simulink model "XFLUID04_reference"  (R2025a)
settings: Solver=ode23t  StartTime=0  StopTime=20  MaxStep=0.02  RelTol=1e-3  AbsTol=1e-4  EnableMultiTasking=on
PreLoadFcn:
  | warning('off','Simulink:Commands:LoadMdlParameterizedLink');
PostLoadFcn:
  | warning off sm:compiler:topologyAnalysis:DanglingBlock
  | warning off Simulink:SL_SolverMaskedZC;
  | warning off Simulink:SL_SolverIgnoredZCBracketing;
  | warning off Simulink:Engine:SolverMinStepNonlinearIterWarnForDAE;
  | warning off simscape:compiler:sli:init:SolverNotRecommended
  | warning off Simulink:Engine:UsingDiscreteSolver
  | warning('off','sm:sli:setup:compile:LocalSolverNotSupported')
  | warning off physmod:simscape:compiler:sli:init:SolverNotRecommended
  | warning off sm:sli:visualization:ModelRefNotSupported
  | warning off Simulink:modelReference:ProtectedModelCallbackLostWarning
StartFcn:
  | tic;
StopFcn:
  | Elapsed_Sim_Time = toc;
  | disp(['Elapsed Sim Time = ' num2str(Elapsed_Sim_Time)]);
undefined symbols (not defined in the file): actuator_hs_b, actuator_hs_k, lift_target_mm, Local, motion_start_s, motor_damping, pressure_step_offset_s, ramp_duration_s, Scissor_Lift_Param, supply_pressure_bar, supply_pressure_step_fraction, target_hold_s, X, Y, Z
libraries: fl_lib x108, sm_lib x41, Scissor_Parts_Lib x24, nesl_utility x9, SimscapeFluids_lib x2, Custom_lib x2, slpidlib x1, fl_ps_legacy_lib x1, simulink x1, ee_lib x1, Motor_Lib x1, sdl_lib x1
(part 1 of 3)
Description:
  | Copyright 2015-2025 The MathWorks, Inc.
settings Model: ExtModeTrigDuration=500  Creator=smiller  LastModifiedBy=SimuVerity Contributors
settings SolverCC: AutoScaleAbsTol=off  AlgebraicLoopSolver=TrustRegion  PositivePriorityOrder=on
settings DataIOCC: SaveFormat=Array
settings OptimizationCC: BlockReduction=off  OptimizeBlockIOStorage=off  BufferReuse=off  ReuseModelBlockBuffer=off  GlobalBufferReuse=off  ExpressionFolding=off  ExpressionDepthLimit=2147483647.0  LocalBlockOutputs=off  ZeroExternalMemoryAtStartup=off  ZeroInternalMemoryAtStartup=off  OptimizeDataStoreBuffers=off  BusAssignmentInplaceUpdate=off
settings DebuggingCC: UnderspecifiedInitializationDetection=Classic  MergeDetectMultiDrivingBlocksExec=none  UnconnectedInputMsg=warning  UnconnectedOutputMsg=warning  UnconnectedLineMsg=warning  AllowSymbolicDim=off  StateNameClashWarn=warning  PregeneratedLibrarySubsystemCodeDiagnostic=none  SFUnexpectedBacktrackingDiag=warning  SFNoUnconditionalDefaultTransitionDiag=warning  SFExecutionAtInitializationDiag=none  ArithmeticOperatorsInVariantConditions=warning
settings ModelReferenceCC: EnableRefExpFcnMdlSchedulingChecks=on  PropagateSignalLabelsOutOfModel=off
settings SFSimCC: SimUseLocalCustomCode=off  CustomCodeUndefinedFunction=UseInterfaceOnly
settings RTWCC: RTWUseLocalCustomCode=off  Toolchain=Simulink Real-Time Toolchain  BuildConfiguration=Faster Runs  TargetLang=C++  GPUComputeCapability=3.5  DLArmComputeVersion=19.05
settings CodeAppCC: StateflowObjectComments=on
settings GRTTargetCC: TargetLangStandard=C++03 (ISO)  CodeInterfacePackaging=C++ class
settings ConfigComp: CovMetricSettings=dw  CovSaveCumulativeToWorkspaceVar=on  CovSaveSingleToWorkspaceVar=on  CovExternalEMLEnable=off  CovSFcnEnable=off
settings SimscapeCC: ExplicitSolverDiagnosticOptions=none  SimscapeNormalizeSystem=off  SimscapeLogType=all  SimscapeLogSimulationStatistics=on  SimscapeLogName=simlog_ssc_hydraulic_lift  SimscapeLogLimitData=off
settings ConfigurationSet: Description=SimMechanics 2G
settings DiagnosticsConfigSet: SimMechanicsUnconnectedFramePorts=none
settings ExplorerConfigSet: SimMechanicsOpenEditorOnUpdate=off  InternalSimMechanicsExplorerSettings="<ExplorerConfiguration><canonicalview>default</canonicalview><AnimationSetting><BasePlaybackSpeed>1.0</BasePlaybackSpeed><PlaybackSpeedFactor>1.0</PlaybackSpeedFactor></AnimationSetting><TilePanel><TileInfo><Tiles Columns=\"1\" Count=\"1\" Rows=\"1\"><Column Left=\"2\" Weight=\"1\"/><Column Left=\"550\"/><Row Top=\"2\" Weight=\"1\"/><Row Top=\"610\"/><Tile Height=\"1\" Width=\"1\" X=\"0\" Y=\"0\"/></Tiles></TileInfo><SceneInfo><SceneViewer><BGColor><R>0.90980392694473267</R><G>1</G><B>1</B></BGColor><Camera><Position><X>-3.0625353892662139</X><Y>-4.5689256897751696</Y><Z>1.9819473078285381</Z></Position><Center><X>-0.9000098372499532</X><Y>-2.432211148661878e-05</Y><Z>1.1621088702953468</Z></Center><Up><X>0.060248240113841743</X><Y>0.14860062570234261</Y><Z>0.98706028367271337</Z></Up><Left>-1.3650000751018525</Left><Right>1.3650000751018525</Right><Bottom>-1.2464621901512147</Bottom><Top>1.2464621901512147</Top></Camera></SceneViewer></SceneInfo></TilePanel></ExplorerConfiguration>"

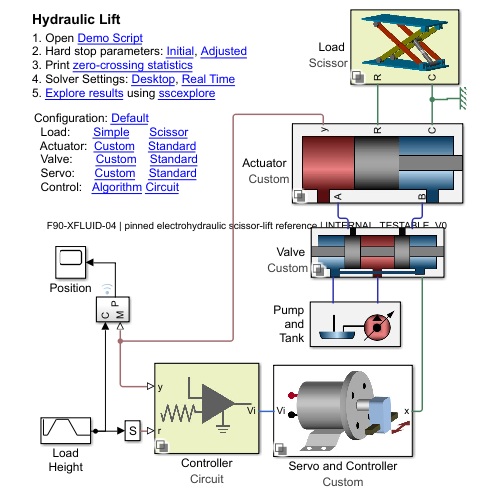
[thumbnail: Simulink's stored preview of the top-level diagram]
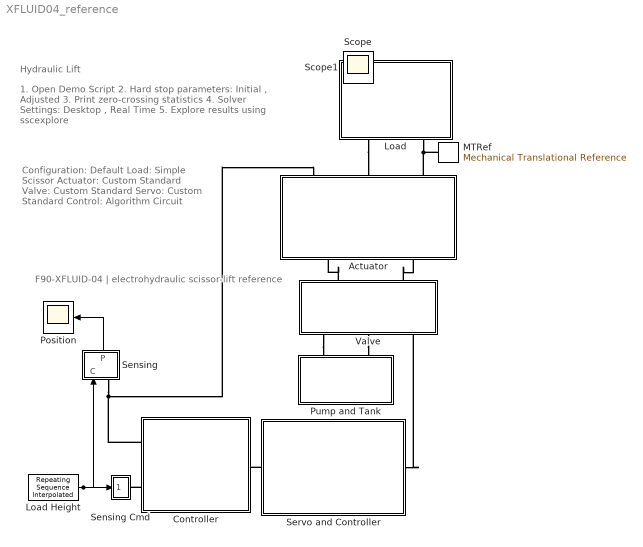
== system XFLUID04_reference ==
  note: Hydraulic Lift
  note: 1. Open Demo Script
      | 2. Hard stop parameters: Initial , Adjusted
      | 3. Print zero-crossing statistics
      | 4. Solver Settings: Desktop , Real Time
      | 5. Explore results using sscexplore
  note: Configuration: Default
      | Load: Simple Scissor
      | Actuator: Custom Standard
      | Valve: Custom Standard
      | Servo: Custom Standard
      | Control: Algorithm Circuit
  note: F90-XFLUID-04 | electrohydraulic scissor-lift reference
  Actuator : Subsystem  Variant=on  VariantControlMode=label  LabelModeActiveChoice=Custom
      settings: AttributesFormatString=%<ActiveVariant>
      mask Display:
      | blk = ssc_hydraulic_lift_activeVariantBlock(gcb);
      | eval(get_param(blk, 'MaskDisplay'));
  Controller : Subsystem  Variant=on  VariantControlMode=label  LabelModeActiveChoice=Circuit
      settings: AttributesFormatString=%<ActiveVariant>
      mask Display:
      | blk = ssc_hydraulic_lift_activeVariantBlock(gcb);
      | eval(get_param(blk, 'MaskDisplay'));
  Load : Subsystem  Variant=on  VariantControlMode=label  LabelModeActiveChoice=Scissor
      settings: AttributesFormatString=%<ActiveVariant>
      mask Display:
      | blk = ssc_hydraulic_lift_activeVariantBlock(gcb);
      | eval(get_param(blk, 'MaskDisplay'));
  Load Height : simulink/Sources/Repeating Sequence Interpolated  OutValues=[2.5 2.5 2.5+(lift_target_mm-50)*Scissor_Lift_Param.Sensor_Gain/1000 2.5+(lift_target_mm-50)*Scissor_Lift_Param.Sensor_Gain/1000 2.5 2.5]  TimeValues=[0 motion_start_s motion_start_s+ramp_duration_s motion_start_s+ramp_duration_s+target_hold_s motion_start_s+2*ramp_duration_s+target_hold_s 20]  LookUpMeth=Interpolation-Use End Values  tsamp=0.01  OutMin=[]  OutMax=[]  OutDataTypeStr=double  OutputDataTypeScalingMode=double  OutDataType=fixdt(0,8)  OutScaling=2^-10
  MTRef : fl_lib/Mechanical/Translational Elements/Mechanical Translational Reference
  Position : Scope
      settings: ActiveDisplayYMinimum=-77.71015  ActiveDisplayYMaximum=177.54113  DataLoggingVariableName=LoadPosition_DATA
  Pump and Tank : Subsystem
      mask Display: image('Pump_IMAGE.jpg');
  Sensing : Subsystem
  Sensing Cmd : Subsystem
      mask Display: disp('S')
  Servo and Controller : Subsystem  Variant=on  VariantControlMode=label  LabelModeActiveChoice=Custom
      settings: AttributesFormatString=%<ActiveVariant>
      mask Display:
      | blk = ssc_hydraulic_lift_activeVariantBlock(gcb);
      | eval(get_param(blk, 'MaskDisplay'));
  Valve : Subsystem  Variant=on  VariantControlMode=label  LabelModeActiveChoice=Custom
      settings: AttributesFormatString=%<ActiveVariant>
      mask Display:
      | blk = ssc_hydraulic_lift_activeVariantBlock(gcb);
      | eval(get_param(blk, 'MaskDisplay'));
  Scope : Scope
      settings: ActiveDisplayYMinimum=-0.84217  ActiveDisplayYMaximum=5.75412
  Scope1 : Scope
      settings: ActiveDisplayYMinimum=-0.31315  ActiveDisplayYMaximum=0.39292  DataLoggingVariableName=ScopeData2
  wires:
  Sensing/1(P) -> Position/1
  Load Height/1 -> Sensing/1(C), Sensing Cmd/1(In1)
  connections:
  MTRef/LConn1 -- Load/LConn2 -- Actuator/RConn3
  Valve/RConn1 -- Actuator/LConn1
  Valve/RConn2 -- Actuator/LConn2
  Controller/LConn1 -- Sensing/LConn1 -- Actuator/RConn1
  Load/LConn1 -- Actuator/RConn2
  Valve/LConn1 -- Pump and Tank/RConn1
  Valve/LConn2 -- Pump and Tank/RConn2
  Servo and Controller/RConn1 -- Valve/LConn3
  Servo and Controller/LConn1 -- Controller/RConn1
  Controller/LConn2 -- Sensing Cmd/RConn1

== system XFLUID04_reference/Actuator ==
  note: Variant Subsystem
  Custom : Subsystem  VariantControl=Custom  mask(Double-Acting Hydraulic Actuator){A=5e-4, V=10e-5, PA=200, PB=0, T=200, hs_k=actuator_hs_k, hs_b=actuator_hs_b}
      mask prompts: A "Piston area (m^2)"; V "Chamber dead volume (m^3)"; PA "Chamber A initial pressure (bar)"; PB "Chamber B initial pressure (bar)"; T "Piston travel (mm)"; hs_k "Hardstop stiffness (N/m)"; hs_b "Hardstop damping (N/(m/s))"
      mask help: Models a double-acting hydraulic actuator using Simscape Foundation library components.
      mask Display: image('Double_Acting_Cylinder_Custom_IMAGE.jpg');
  Standard : Subsystem  VariantControl=Standard  mask(Double-Acting Hydraulic Actuator){A=5e-4, V=10e-5, PA=200, PB=0, T=200, hs_k=actuator_hs_k, hs_b=actuator_hs_b}
      mask prompts: A "Piston area (m^2)"; V "Chamber dead volume (m^3)"; PA "Chamber A initial pressure (bar)"; PB "Chamber B initial pressure (bar)"; T "Piston travel (mm)"; hs_k "Hardstop stiffness (N/m)"; hs_b "Hardstop damping (N/(m/s))"
      mask help: Models a double-acting hydraulic actuator using Simscape add-on library components.
      mask Display: image('Double_Acting_Cylinder_Standard_IMAGE.jpg');
  A : PMIOPort  Side=Left
  B : PMIOPort  Port=2  Side=Left
  y : PMIOPort  Port=3  Side=Right
  R : PMIOPort  Port=4  Side=Right
  C : PMIOPort  Port=5  Side=Right

== system XFLUID04_reference/Controller ==
  Algorithm : Subsystem  VariantControl=Algorithm
      mask Display: image('Algorithm_Controller_IMAGE.jpg')
  Circuit : Subsystem  VariantControl=Circuit
      mask Display: image('Analog_PI_Controller_IMAGE.jpg')
  y : PMIOPort  Tag=PMCPort  Side=Left
  r : PMIOPort  Tag=PMCPort  Port=2  Side=Left
  Vi : PMIOPort  Port=3  Side=Right

== system XFLUID04_reference/Load ==
  Scissor : Subsystem  VariantControl=Scissor
      mask Display: image('Load_Scissor_IMAGE.jpg');
  Simple : Subsystem  VariantControl=Simple
      mask Display: image('Load_Simple_IMAGE.jpg');
  R : PMIOPort  Side=Left
  C : PMIOPort  Port=2  Side=Left

== system XFLUID04_reference/Pump and Tank ==
  Custom Hydraulic Fluid : fl_lib/Isothermal Liquid/Utilities/Isothermal Liquid Properties (IL)  rho_L_atm=850 kg/m^3  bulk_modulus_model=foundation.enum.bulk_modulus_model.const  beta_gain=6  beta_L_atm=8e+08 Pa  nu_atm=1.8e-05 m^2/s  p_atm=0.101325 MPa  p_min=1 Pa  properties_range_check=simscape.enum.assert.action.error  air_fraction=0.005  polytropic_index=1.0  rho_g_atm=1.225 kg/m^3  air_dissolution_model=false  p_crit=3 MPa
      settings: LibrarySourceBlock=fl_lib/Isothermal Liquid/Utilities/Isothermal Liquid Properties (IL)
  Hydraulic Reference : fl_lib/Isothermal Liquid/Elements/Reservoir (IL)  reservoir_type=foundation.enum.constant_controlled.constant  pressure_spec=foundation.enum.pressure_spec.atmospheric  reservoir_pressure=0.101325 MPa
  Pump : fl_lib/Isothermal Liquid/Sources/Pressure Source (IL)  source_type=foundation.enum.constant_controlled.controlled  pressure_differential=0 MPa
      settings: InternalSimscapePortConfiguration="{\"Bottom\":[],\"Left\":[{\"id\":\"A\",\"label\":\"A\",\"type\":\"foundation.isothermal_liquid.isothermal_liquid\"},{\"id\":\"P\",\"label\":\"P\",\"type\":\"input\"}],\"Right\":[{\"id\":\"B\",\"label\":\"B\",\"type\":\"foundation.isothermal_liquid.isothermal_liquid\"}],\"Top\":[]}"
  Solver Configuration : nesl_utility/Solver Configuration  PhysicalDomain=network_engine_domain  SubClassName=solver  LeftPortType=input  RightPortType=generic  Tones=[]  Harmonics=[]  SimulateNoise=off  Profile=off  UseLocalSampling=off  EnableSwitchedLinearOptims=on  FrequencyDomain=off  UseCCode=off  RelTol=0.001  AbsTol=1e-06  MinStep=1e-09  ToWorkspace=off  RevertToSquareIcSolve=off  NumHomotopyIterations=100  PhasorMode=off  PhasorModeNumHarmonics=1  ConsistencySolver=NEWTON_FTOL  IndexReductionMethod=DerivativeReplacement  DoDC=off  ResidualTolerance=1e-9  ConsistencyTolSource=GLOBAL  ConsistencyAbsTol=0.001  ConsistencyRelTol=0.001  ConsistencyTolFactor=0.001  UseLocalSolver=off  LocalSolverChoice=NE_BACKWARD_EULER_ADVANCER  ResolveIndetEquations=on  FunctionEvalNumThread=1  LocalSolverSampleTime=0.002  DoFixedCost=off  MaxNonlinIter=4  MaxModeIter=2  ComputeImpulses=off  ImpulseIterations=2  LinearAlgebra=Sparse  LinearAlgebraNumThread=0  EquationFormulation=NE_TIME_EF  DelaysMemoryBudget=1024  AutomaticFiltering=on  FilteringTimeConstant=0.001  PartitionStorageMethod=AS_NEEDED  PartitionMemoryBudget=1024  PartitionMethod=FAST  MultibodyUseLocalSolver=off  MultibodyLocalSolverChoice=ODE1  MultibodyLocalSolverSampleTime=0.001
  Supply Pressure : Step  Time=motion_start_s+ramp_duration_s+pressure_step_offset_s  Before=supply_pressure_bar  After=supply_pressure_bar*(1+supply_pressure_step_fraction)  SampleTime=0
  bar : nesl_utility/Simulink-PS Converter  PhysicalDomain=network_engine_domain  SubClassName=ps_input  LeftPortType=input  RightPortType=output  PseudoPeriodic=off  Frequencies=[]  NoiseDistribution=none  NoiseParameters=[]  Unit=bar  AffineConversion=off  FilteringAndDerivatives=zero  SimscapeFilterOrder=1  InputFilterTimeConstant=0.005  UdotUserProvided=0
  T : PMIOPort  Side=Right
  P : PMIOPort  Port=2  Side=Right
  wires:
  Supply Pressure/1 -> bar/1
  connections:
  Custom Hydraulic Fluid/RConn1 -- Solver Configuration/RConn1 -- T/RConn1 -- Pump/LConn1 -- Hydraulic Reference/LConn1
  P/RConn1 -- Pump/RConn1
  bar/RConn1 -- Pump/LConn2

== system XFLUID04_reference/Sensing ==
  C : Inport
  Fcn : Fcn  Expr=(u(1)-2.5)*1000/Scissor_Lift_Param.Sensor_Gain+50
  Mux : Mux  Inputs=2
  PS-Simulink Converter : nesl_utility/PS-Simulink Converter  PhysicalDomain=network_engine_domain  SubClassName=ps_output  LeftPortType=input  RightPortType=output  PseudoPeriodic=off  Frequencies=[]  VectorFormat=1-D array  Unit=mm  AffineConversion=off
  M : PMIOPort  Side=Left
  P : Outport  VectorParamsAs1DForOutWhenUnconnected=off
  wires:
  PS-Simulink Converter/1 -> Mux/2
  Mux/1 -> P/1
  Fcn/1 -> Mux/1
  C/1 -> Fcn/1
  connections:
  PS-Simulink Converter/LConn1 -- M/RConn1

== system XFLUID04_reference/Sensing Cmd ==
  In1 : Inport
  Simulink-PS Converter : nesl_utility/Simulink-PS Converter  PhysicalDomain=network_engine_domain  SubClassName=ps_input  LeftPortType=input  RightPortType=output  PseudoPeriodic=off  Frequencies=[]  NoiseDistribution=none  NoiseParameters=[]  Unit=V  AffineConversion=off  FilteringAndDerivatives=filter  SimscapeFilterOrder=1  InputFilterTimeConstant=0.005  UdotUserProvided=1
  Conn1 : PMIOPort  Side=Right
  wires:
  In1/1 -> Simulink-PS Converter/1
  connections:
  Simulink-PS Converter/RConn1 -- Conn1/RConn1

== system XFLUID04_reference/Servo and Controller ==
  note: Variant Subsystem
  Custom : Subsystem  VariantControl=Custom  mask(Servo and controller){G=0.5e-3/(pi/2), x_max=0.5, J=1e-4, lambda=motor_damping, R=10, L=2.5, Kt=0.04, R_controller=[10e3 10e3 10e3 100e3 50 100e3 10e3]}
      mask prompts: G "Spool travel per rotation (m)"; x_max "Spool travel limit (mm)"; J "Shaft inertia (kg m^2)"; lambda "Shaft damping (Nm/(rad/s))"; R "Winding resistance (ohms)"; L "Winding inductance (H)"; Kt "Torque constant (Nm/A)"; R_controller "[R1 R2 R3 R4 R5 R6 R7] (ohms)"
      mask help: Models a servomotor and controller using Simscape Foundation library components.
      mask DialogControl DescTextVar_copy Prompt: Controller resistance values
      mask Display: image('DC_Motor_Custom_IMAGE.jpg')
  Standard : Subsystem  VariantControl=Standard  mask(Servo and controller){G=0.5e-3/(pi/2), x_max=0.5, J=1e-4, lambda=motor_damping, R=10, L=2.5, Kt=0.04, R_controller=[10e3 10e3 10e3 100e3 50 100e3 10e3]}
      mask prompts: G "Spool travel per rotation (m)"; x_max "Spool travel limit (mm)"; J "Shaft inertia (kg m^2)"; lambda "Shaft damping (Nm/(rad/s))"; R "Winding resistance (ohms)"; L "Winding inductance (H)"; Kt "Torque constant (Nm/A)"; R_controller "[R1 R2 R3 R4 R5 R6 R7] (ohms)"
      mask help: Models a servomotor and controller using Simscape add-on library components.
      mask DialogControl DescTextVar_copy Prompt: Controller resistance values
      mask Display: image('DC_Motor_Standard_IMAGE.jpg')
  Vi : PMIOPort  Side=Left
  x : PMIOPort  Port=2  Side=Right

== system XFLUID04_reference/Valve ==
  note: Variant Subsystem
  Custom : Subsystem  VariantControl=Custom  mask(Single-Stage Servo Valve){K_V=0.5, x_max=0.5, A_max=9, x_lap=0.02, A_leak=0.25}
      mask prompts: K_V "Flow Coefficient:"; x_max "Spool travel limit (mm)"; A_max "Maximum orifice area (mm^2)"; x_lap "Spool travel with leakage (mm)"; A_leak "Leakage area at x=0 (mm^2)"
      mask help: Models a spool valve actuated directly by a torque motor using Simscape Foundation library components.
      mask Display: image('Four_Way_Valve_Custom_IMAGE.jpg')
  Standard : Subsystem  VariantControl=Standard  mask(Single-Stage Servo Valve){K_V=0.5, x_max=0.5, A_max=9, x_lap=0.02, A_leak=0.25}
      mask prompts: K_V "Flow Coefficient:"; x_max "Spool travel limit (mm)"; A_max "Maximum orifice area (mm^2)"; x_lap "Spool travel with leakage (mm)"; A_leak "Leakage area at x=0 (mm^2)"
      mask help: Models a spool valve actuated directly by a torque motor using Simscape add-on library components.
      mask Display: image(imread('Four_Way_Valve_Standard_IMAGE.jpg'))
  T : PMIOPort  Tag=PMCPort  Side=Left
  P : PMIOPort  Tag=PMCPort  Port=2  Side=Left
  x : PMIOPort  Tag=PMCPort  Port=3  Side=Left
  A : PMIOPort  Tag=PMCPort  Port=4  Side=Right
  B : PMIOPort  Tag=PMCPort  Port=5  Side=Right

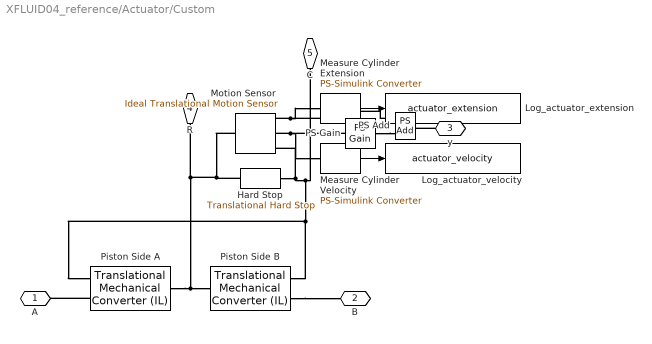
== system XFLUID04_reference/Actuator/Custom ==
  " Motion Sensor" : fl_lib/Mechanical/Mechanical Sensors/Ideal Translational Motion Sensor  reference=foundation.enum.MeasurementReference.difference  acceleration_port=false  velocity_port=true  position_port=true  offset=Scissor_Lift_Param.Initial_Cyl_Ext mm
  Hard Stop : fl_lib/Mechanical/Translational Elements/Translational Hard Stop  upper_bnd=T/2 mm  lower_bnd=-T/2 mm  model=3  stiff_up=hs_k N/m  stiff_low=hs_k N/m  D_up=hs_b N/(m/s)  D_low=hs_b N/(m/s)  transition=0.1 mm  coeff_rest=0.7  v_tol=0.001 m/s  f_tol=0.001 N  v_specify=off  v_priority=High  v=0 m/s  v_nominal_specify=off  v_nominal_value=1  v_nominal_unit=m/s  f_specify=off  f_priority=High  f=0 N  f_nominal_specify=off  f_nominal_value=1  f_nominal_unit=N  x_specify=on  x_priority=High  x=0 m  x_nominal_specify=off  x_nominal_value=1  x_nominal_unit=m  M_specify=off  M_priority=None  M=0
  Log_actuator_extension : ToWorkspace  VariableName=actuator_extension  SaveFormat=Timeseries  SampleTime=-1
  Log_actuator_velocity : ToWorkspace  VariableName=actuator_velocity  SaveFormat=Timeseries  SampleTime=-1
  Measure Cylinder Extension : nesl_utility/PS-Simulink Converter  PhysicalDomain=network_engine_domain  SubClassName=ps_output  LeftPortType=input  RightPortType=output  PseudoPeriodic=off  Frequencies=[]  VectorFormat=inherit  Unit=mm  AffineConversion=off
  Measure Cylinder Velocity : nesl_utility/PS-Simulink Converter  PhysicalDomain=network_engine_domain  SubClassName=ps_output  LeftPortType=input  RightPortType=output  PseudoPeriodic=off  Frequencies=[]  VectorFormat=inherit  Unit=mm/s  AffineConversion=off
  PS Add : fl_lib/Physical Signals/Functions/PS Add
  PS Gain : fl_lib/Physical Signals/Functions/PS Gain  gain=0.1 s
  Piston Side A : fl_lib/Isothermal Liquid/Elements/Translational Mechanical Converter (IL)  mech_orientation=1  displacement_spec=foundation.enum.DisplacementSpec.Calculate  x0=0 m  interface_area=A m^2  dead_volume=V m^3  pressure_spec=1  environment_pressure=0.101325 MPa  dynamic_compressibility=true  p0=0 + 101325 Pa  p_nominal=0.101325 MPa
      settings: LibrarySourceBlock=fl_lib/Isothermal Liquid/Elements/Translational Mechanical Converter (IL)  InternalSimscapePortConfiguration="{\"Bottom\":[],\"Left\":[{\"id\":\"A\",\"label\":\"A\",\"type\":\"foundation.isothermal_liquid.isothermal_liquid\"},{\"id\":\"C\",\"label\":\"C\",\"type\":\"foundation.mechanical.translational.translational\"}],\"Right\":[{\"id\":\"R\",\"label\":\"R\",\"type\":\"foundation.mechanical.translational.translational\"}],\"Top\":[]}"
  Piston Side B : fl_lib/Isothermal Liquid/Elements/Translational Mechanical Converter (IL)  mech_orientation=-1  displacement_spec=foundation.enum.DisplacementSpec.Calculate  x0=-(0) m  interface_area=A m^2  dead_volume=V m^3  pressure_spec=1  environment_pressure=0.101325 MPa  dynamic_compressibility=true  p0=0 + 101325 Pa  p_nominal=0.101325 MPa
      settings: LibrarySourceBlock=fl_lib/Isothermal Liquid/Elements/Translational Mechanical Converter (IL)  InternalSimscapePortConfiguration="{\"Bottom\":[],\"Left\":[{\"id\":\"A\",\"label\":\"A\",\"type\":\"foundation.isothermal_liquid.isothermal_liquid\"},{\"id\":\"C\",\"label\":\"C\",\"type\":\"foundation.mechanical.translational.translational\"}],\"Right\":[{\"id\":\"R\",\"label\":\"R\",\"type\":\"foundation.mechanical.translational.translational\"}],\"Top\":[]}"
  A : PMIOPort  Side=Left
  B : PMIOPort  Port=2  Side=Left
  y : PMIOPort  Port=3  Side=Right
  R : PMIOPort  Port=4  Side=Right
  C : PMIOPort  Port=5  Side=Right
  wires:
  Measure Cylinder Extension/1 -> Log_actuator_extension/1
  Measure Cylinder Velocity/1 -> Log_actuator_velocity/1
  connections:
  " Motion Sensor"/RConn3 -- PS Add/LConn1 -- Measure Cylinder Extension/LConn1
  Hard Stop/RConn1 -- " Motion Sensor"/RConn1 -- Piston Side A/LConn2 -- Piston Side B/LConn2 -- C/RConn1
  Piston Side A/LConn1 -- A/RConn1
  Piston Side B/LConn1 -- B/RConn1
  " Motion Sensor"/RConn2 -- PS Gain/LConn1 -- Measure Cylinder Velocity/LConn1
  y/RConn1 -- PS Add/RConn1
  PS Gain/RConn1 -- PS Add/LConn2
  " Motion Sensor"/LConn1 -- Piston Side A/RConn1 -- Piston Side B/RConn1 -- R/RConn1 -- Hard Stop/LConn1

== system XFLUID04_reference/Actuator/Standard ==
  " Motion Sensor" : fl_lib/Mechanical/Mechanical Sensors/Ideal Translational Motion Sensor  reference=foundation.enum.MeasurementReference.difference  acceleration_port=false  velocity_port=true  position_port=true  offset=Scissor_Lift_Param.Initial_Cyl_Ext mm
  Double-Acting Hydraulic Cylinder : SimscapeFluids_lib/Isothermal Liquid/Actuators/Double-Acting Actuator (IL)  single_fluid=true  mech_orientation=1  piston_area_A=A m^2  piston_area_B=A m^2  stroke=T mm  dead_volume_A=V m^3  dead_volume_B=V m^3  pressure_spec=foundation.enum.pressure_spec.atmospheric  environment_pressure=0.101325 MPa  hardstop_model=3  stiff_coeff=hs_k N/m  damping_coeff=hs_b N/(m/s)  transition=0.1 mm  coeff_rest=0.7  v_tol=0.001 m/s  f_tol=0.001 N  cushion_A_spec=false  area_plunger_A=1e-4 m^2  length_plunger_A=1e-3 m  area_cushion_orifice_A=1e-6 m^2  area_leak_plunger_A=1e-7 m^2  p_crack_differential_A=0.01 MPa  press_max_differential_A=0.1 MPa  check_valve_area_max_A=1e-4 m^2  check_valve_area_leak_A=1e-10 m^2  smoothing_factor_A=0  cushion_B_spec=false  area_plunger_B=1e-4 m^2  length_plunger_B=1e-3 m  area_cushion_orifice_B=1e-6 m^2  area_leak_plunger_B=1e-7 m^2  p_crack_differential_B=0.01 MPa  press_max_differential_B=0.1 MPa  check_valve_area_max_B=1e-4 m^2  check_valve_area_leak_B=1e-10 m^2  smoothing_factor_B=0  friction_spec=false  breakaway_Coulomb_ratio=1.2  breakaway_velocity=0.1 m/s  preload_force=20 N  Coulomb_coeff=1e-6 N/Pa  viscous_coeff=100 N*s/m  leakage_spec=false  clearance=1e-4 m  piston_length=0.01 m  displacement_spec=foundation.enum.DisplacementSpec.Calculate  x0=T/2 mm  dynamic_compressibility=true  p0_A=PA + 1.01325 bar  p0_B=PB + 1.01325 bar  p_nominal_A=0.101325 MPa  p_nominal_B=0.101325 MPa
      settings: LibrarySourceBlock=SimscapeFluids_lib/Isothermal Liquid/Actuators/Double-Acting Actuator (IL)  InternalSimscapePortConfiguration="{\"Bottom\":[],\"Left\":[{\"id\":\"C\",\"label\":\"C\",\"type\":\"foundation.mechanical.translational.translational\"},{\"id\":\"A\",\"label\":\"A\",\"type\":\"foundation.isothermal_liquid.isothermal_liquid\"}],\"Right\":[{\"id\":\"p_out\",\"label\":\"p\",\"type\":\"output\"},{\"id\":\"R\",\"label\":\"R\",\"type\":\"foundation.mechanical.translational.translational\"},{\"id\":\"B\",\"label\":\"B\",\"type\":\"foundation.isothermal_liquid.isothermal_liquid\"}],\"Top\":[]}"
  PS Add : fl_lib/Physical Signals/Functions/PS Add
  PS Gain : fl_lib/Physical Signals/Functions/PS Gain  gain=0.1 s
  A : PMIOPort  Side=Left
  B : PMIOPort  Port=2  Side=Left
  y : PMIOPort  Port=3  Side=Right
  R : PMIOPort  Port=4  Side=Right
  C : PMIOPort  Port=5  Side=Right
  connections:
  y/RConn1 -- PS Add/RConn1
  C/RConn1 -- Double-Acting Hydraulic Cylinder/LConn1 -- " Motion Sensor"/RConn1
  Double-Acting Hydraulic Cylinder/RConn3 -- B/RConn1
  PS Gain/RConn1 -- PS Add/LConn2
  " Motion Sensor"/RConn2 -- PS Gain/LConn1
  PS Add/LConn1 -- " Motion Sensor"/RConn3
  " Motion Sensor"/LConn1 -- R/RConn1 -- Double-Acting Hydraulic Cylinder/RConn2
  A/RConn1 -- Double-Acting Hydraulic Cylinder/LConn2

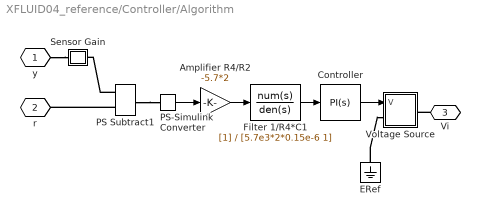
== system XFLUID04_reference/Controller/Algorithm ==
  Amplifier R4/R2 : Gain  Gain=-5.7*2
  Controller : slpidlib/PID Controller  Controller=PI  Form=Parallel  TimeDomain=Continuous-time  UseExternalTs=off  SampleTime=-1  IntegratorMethod=Forward Euler  FilterMethod=Forward Euler  ControllerParametersSource=internal  P=20/10  I=1/(10e3*100e-6*100)  UseKiTs=off  D=0  UseExternalDerivativeSource=off  N=100  UseFilter=on  TunerSelectOption=Transfer Function Based (PID Tuner App)  InitialConditionSource=internal  InitialConditionForIntegrator=0  InitialConditionForFilter=0  DifferentiatorICPrevScaledInput=0  ExternalReset=none  TrackingMode=off  Kt=1  LimitOutput=off  SatLimitsSource=internal  UpperSaturationLimit=inf  LowerSaturationLimit=-inf  LinearizeAsGain=on  AntiWindupMode=none  Kb=1  LimitIntegrator=off  UpperIntegratorSaturationLimit=inf  LowerIntegratorSaturationLimit=-inf  POutMin=[]  POutMax=[]  IOutMin=[]  IOutMax=[]  DOutMin=[]  DOutMax=[]  NOutMin=[]  NOutMax=[]  SumOutMin=[]  SumOutMax=[]  SaturationOutMin=[]  SaturationOutMax=[]  PParamMin=[]  PParamMax=[]  IParamMin=[]  IParamMax=[]  DParamMin=[]  DParamMax=[]  NParamMin=[]  NParamMax=[]  KbParamMin=[]  KbParamMax=[]  KtParamMin=[]  KtParamMax=[]  KbOutMin=[]  KbOutMax=[]  KtOutMin=[]  KtOutMax=[]  IntegratorOutMin=[]  IntegratorOutMax=[]  FilterOutMin=[]  FilterOutMax=[]  SumI1OutMin=[]  SumI1OutMax=[]  SumI2OutMin=[]  SumI2OutMax=[]  SumI3OutMin=[]  SumI3OutMax=[]  SumI4OutMin=[]  SumI4OutMax=[]  SumDOutMin=[]  SumDOutMax=[]  DifferentiatorOutMin=[]  DifferentiatorOutMax=[]  FilterDiffOutCoefMin=[]  FilterDiffOutCoefMax=[]  ReciprocalOutMin=[]  ReciprocalOutMax=[]  SumDenOutMin=[]  SumDenOutMax=[]  SumNumOutMin=[]  SumNumOutMax=[]  DivideOutMin=[]  DivideOutMax=[]  UdiffTsProdOutMin=[]  UdiffTsProdOutMax=[]  NTsProdOutMin=[]  NTsProdOutMax=[]  UintegralTsProdOutMin=[]  UintegralTsProdOutMax=[]  UngainTsProdOutMin=[]  UngainTsProdOutMax=[]  ClampingZeroOutDataTypeStr=Inherit: Inherit via back propagation  ClampingZeroOutMin=[]  ClampingZeroOutMax=[]  FilterDenConstantOutDataTypeStr=Inherit: Inherit via back propagation  FilterDenConstantOutMin=[]  FilterDenConstantOutMax=[]  PCopyOutDataTypeStr=Inherit: Inherit via back propagation  PCopyOutMin=[]  PCopyOutMax=[]  NCopyOutDataTypeStr=Inherit: Inherit via back propagation  NCopyOutMin=[]  NCopyOutMax=[]  IntegratorContinuousStateAttributes=''  IntegratorStateMustResolveToSignalObject=off  IntegratorRTWStateStorageClass=Auto  FilterContinuousStateAttributes=''  FilterStateMustResolveToSignalObject=off  FilterRTWStateStorageClass=Auto  ParallelPVariant=InternalParameters  IdealPVariant=Disabled  IVariant=InternalParameters  DVariant=Disabled  IntegratorVariant=Continuous  SatVariant=Disabled  AWVariant=Passthrough  PCopyVariant=Disabled  TRVariant=Disabled  FdbkBlocksVariant=Forward  IdealPFdbkVariant=Disabled  SatFdbkVariant=Disabled  DerivativeFilterVariant=Disabled  NVariant=Disabled  NCopyVariant=Disabled_SignalSpec  FilterICVariant=Disabled  IntegratorICVariant=InternalICs  ExternalResetVariant=Disabled  TRSumVariant=Passthrough  SumFdbkVariant=Disabled  SumVariant=Sum_PI  TsampFilterVariant=InternalTs  TsampNgainVariant=Passthrough  TsampIntegralVariant=Disabled_SignalSpec  ExternalSaturationOutDataTypeStr=Inherit: Same as second input  DerivativeSourceVariant=Disabled  PreIntVariant=InternalPreInt
  ERef : fl_lib/Electrical/Electrical Elements/Electrical Reference
  Filter 1/R4*C1 : TransferFcn  Denominator=[5.7e3*2*0.15e-6 1]
  PS Subtract1 : fl_lib/Physical Signals/Functions/PS Subtract
  PS-Simulink Converter : nesl_utility/PS-Simulink Converter  PhysicalDomain=network_engine_domain  SubClassName=ps_output  LeftPortType=input  RightPortType=output  PseudoPeriodic=off  Frequencies=[]  VectorFormat=1-D array  Unit=V  AffineConversion=off
  Sensor Gain : Subsystem
      mask Display: disp('G')
  Voltage Source : Subsystem
  y : PMIOPort  Tag=PMCPort  Side=Left
  r : PMIOPort  Tag=PMCPort  Port=2  Side=Left
  Vi : PMIOPort  Port=3  Side=Right
  wires:
  PS-Simulink Converter/1 -> Amplifier R4/R2/1
  Amplifier R4/R2/1 -> Filter 1/R4*C1/1
  Filter 1/R4*C1/1 -> Controller/1
  Controller/1 -> Voltage Source/1(V)
  connections:
  PS Subtract1/RConn1 -- PS-Simulink Converter/LConn1
  ERef/LConn1 -- Voltage Source/LConn1
  PS Subtract1/LConn2 -- r/RConn1
  y/RConn1 -- Sensor Gain/LConn1
  Vi/RConn1 -- Voltage Source/RConn1
  PS Subtract1/LConn1 -- Sensor Gain/RConn1

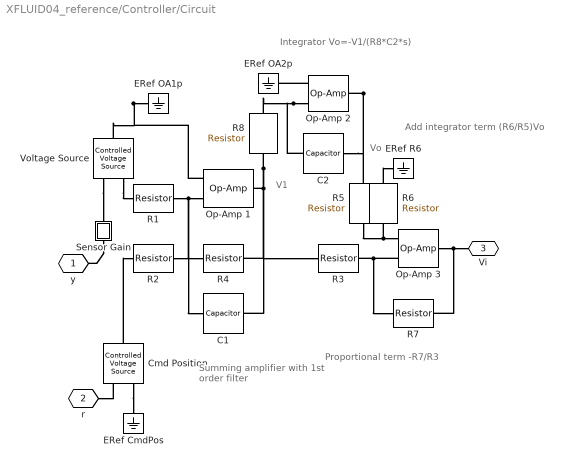
== system XFLUID04_reference/Controller/Circuit ==
  note: V1
  note: Vo
  note: Add integrator
      | term (R6/R5)Vo
  note: Proportional
      | term -R7/R3
  note: Integrator
      | Vo=-V1/(R8*C2*s)
  note: Summing amplifier
      | with 1st order filter
  C1 : fl_lib/Electrical/Electrical Elements/Capacitor  c=0.15e-06 F  r=1e-06 Ohm  g=0 1/Ohm  i_specify=off  i_priority=High  i=0 A  i_nominal_specify=off  i_nominal_value=1  i_nominal_unit=A  v_specify=off  v_priority=High  v=0 V  v_nominal_specify=off  v_nominal_value=1  v_nominal_unit=V  vc_specify=on  vc_priority=High  vc=0 V  vc_nominal_specify=off  vc_nominal_value=1  vc_nominal_unit=V
  C2 : fl_lib/Electrical/Electrical Elements/Capacitor  c=100e-06*100 F  r=1e-06 Ohm  g=0 1/Ohm  i_specify=off  i_priority=High  i=0 A  i_nominal_specify=off  i_nominal_value=1  i_nominal_unit=A  v_specify=off  v_priority=High  v=0 V  v_nominal_specify=off  v_nominal_value=1  v_nominal_unit=V  vc_specify=on  vc_priority=High  vc=0 V  vc_nominal_specify=off  vc_nominal_value=1  vc_nominal_unit=V
  Cmd Position : fl_lib/Electrical/Electrical Sources/Controlled Voltage Source
  ERef CmdPos : fl_lib/Electrical/Electrical Elements/Electrical Reference
  ERef OA1p : fl_lib/Electrical/Electrical Elements/Electrical Reference
  ERef OA2p : fl_lib/Electrical/Electrical Elements/Electrical Reference
  ERef R6 : fl_lib/Electrical/Electrical Elements/Electrical Reference
  Op-Amp 1 : fl_lib/Electrical/Electrical Elements/Op-Amp  outI_specify=off  outI_priority=High  outI=0 A  outI_nominal_specify=off  outI_nominal_value=1  outI_nominal_unit=A
  Op-Amp 2 : fl_lib/Electrical/Electrical Elements/Op-Amp  outI_specify=off  outI_priority=High  outI=0 A  outI_nominal_specify=off  outI_nominal_value=1  outI_nominal_unit=A
  Op-Amp 3 : fl_lib/Electrical/Electrical Elements/Op-Amp  outI_specify=off  outI_priority=High  outI=0 A  outI_nominal_specify=off  outI_nominal_value=1  outI_nominal_unit=A
  R{1..3,5..6,8} (6 alike) : fl_lib/Electrical/Electrical Elements/Resistor  R=10e3 Ohm  i_specify=off  i_priority=High  i=0 A  i_nominal_specify=off  i_nominal_value=1  i_nominal_unit=A  v_specify=off  v_priority=High  v=0 V  v_nominal_specify=off  v_nominal_value=1  v_nominal_unit=V
  R4 : fl_lib/Electrical/Electrical Elements/Resistor  R=5.7e3*2 Ohm  i_specify=off  i_priority=High  i=0 A  i_nominal_specify=off  i_nominal_value=1  i_nominal_unit=A  v_specify=off  v_priority=High  v=0 V  v_nominal_specify=off  v_nominal_value=1  v_nominal_unit=V
  R7 : fl_lib/Electrical/Electrical Elements/Resistor  R=20e3 Ohm  i_specify=off  i_priority=High  i=0 A  i_nominal_specify=off  i_nominal_value=1  i_nominal_unit=A  v_specify=off  v_priority=High  v=0 V  v_nominal_specify=off  v_nominal_value=1  v_nominal_unit=V
  Sensor Gain : Subsystem
      mask Display: disp('G')
  Voltage Source : fl_lib/Electrical/Electrical Sources/Controlled Voltage Source
  y : PMIOPort  Tag=PMCPort  Side=Left
  r : PMIOPort  Tag=PMCPort  Port=2  Side=Left
  Vi : PMIOPort  Port=3  Side=Right
  connections:
  Sensor Gain/LConn1 -- y/RConn1
  Voltage Source/RConn1 -- Sensor Gain/RConn1
  Op-Amp 2/LConn1 -- ERef OA2p/LConn1
  R6/RConn1 -- ERef R6/LConn1
  Cmd Position/RConn2 -- ERef CmdPos/LConn1
  Cmd Position/LConn1 -- R2/LConn1
  Voltage Source/RConn2 -- R1/LConn1
  R3/RConn1 -- R7/LConn1 -- Op-Amp 3/LConn2
  Op-Amp 3/LConn1 -- R6/LConn1 -- R5/RConn1
  ERef OA1p/LConn1 -- Voltage Source/LConn1 -- Op-Amp 1/LConn1
  Op-Amp 2/RConn1 -- R5/LConn1 -- C2/RConn1
  Op-Amp 2/LConn2 -- C2/LConn1 -- R8/RConn1
  R8/LConn1 -- Op-Amp 1/RConn1 -- R3/LConn1 -- C1/RConn1 -- R4/RConn1
  Op-Amp 1/LConn2 -- C1/LConn1 -- R4/LConn1 -- R2/RConn1 -- R1/RConn1
  Op-Amp 3/RConn1 -- R7/RConn1 -- Vi/RConn1
  r/RConn1 -- Cmd Position/RConn1

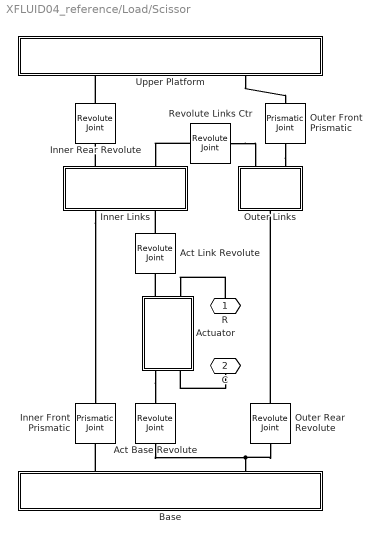
== system XFLUID04_reference/Load/Scissor ==
  Act Base Revolute : sm_lib/Joints/Revolute Joint  JointMode=Normal  CompositeWrenchDir=FollowerOnBase  CompositeWrenchFrame=BaseFrame  SenseConstraintForce=off  SenseConstraintTorque=off  SenseTotalForce=off  SenseTotalTorque=off  PositionTargetSpecify=off  PositionTargetPriority=High  PositionTargetValue=0  PositionTargetValueUnits=deg  VelocityTargetSpecify=off  VelocityTargetPriority=High  VelocityTargetValue=0  VelocityTargetValueUnits=deg/s  EquilibriumPosition=0  EquilibriumPositionUnits=deg  SpringStiffness=0  SpringStiffnessUnits=N*m/deg  DampingCoefficient=0  DampingCoefficientUnits=N*m/(deg/s)  LowerLimitSpecify=off  LowerLimitBound=-90  LowerLimitBoundUnits=deg  LowerLimitStiffness=1e4  LowerLimitStiffnessUnits=N*m/deg  LowerLimitDamping=10  LowerLimitDampingUnits=N*m/(deg/s)  LowerLimitTransitionRegionWidth=0.1  LowerLimitTransitionRegionWidthUnits=deg  UpperLimitSpecify=off  UpperLimitBound=90  UpperLimitBoundUnits=deg  UpperLimitStiffness=1e4  UpperLimitStiffnessUnits=N*m/deg  UpperLimitDamping=10  UpperLimitDampingUnits=N*m/(deg/s)  UpperLimitTransitionRegionWidth=0.1  UpperLimitTransitionRegionWidthUnits=deg  TorqueActuationMode=NoTorque  MotionActuationMode=ComputedMotion  SensePosition=off  SenseVelocity=off  SenseAcceleration=off  SenseTorqueForce=off  SenseLowerLimitTorqueForce=off  SenseUpperLimitTorqueForce=off
  Act Link Revolute : sm_lib/Joints/Revolute Joint  JointMode=Normal  CompositeWrenchDir=FollowerOnBase  CompositeWrenchFrame=BaseFrame  SenseConstraintForce=off  SenseConstraintTorque=off  SenseTotalForce=off  SenseTotalTorque=off  PositionTargetSpecify=off  PositionTargetPriority=High  PositionTargetValue=0  PositionTargetValueUnits=deg  VelocityTargetSpecify=off  VelocityTargetPriority=High  VelocityTargetValue=0  VelocityTargetValueUnits=deg/s  EquilibriumPosition=0  EquilibriumPositionUnits=deg  SpringStiffness=0  SpringStiffnessUnits=N*m/deg  DampingCoefficient=0  DampingCoefficientUnits=N*m/(deg/s)  LowerLimitSpecify=off  LowerLimitBound=-90  LowerLimitBoundUnits=deg  LowerLimitStiffness=1e4  LowerLimitStiffnessUnits=N*m/deg  LowerLimitDamping=10  LowerLimitDampingUnits=N*m/(deg/s)  LowerLimitTransitionRegionWidth=0.1  LowerLimitTransitionRegionWidthUnits=deg  UpperLimitSpecify=off  UpperLimitBound=90  UpperLimitBoundUnits=deg  UpperLimitStiffness=1e4  UpperLimitStiffnessUnits=N*m/deg  UpperLimitDamping=10  UpperLimitDampingUnits=N*m/(deg/s)  UpperLimitTransitionRegionWidth=0.1  UpperLimitTransitionRegionWidthUnits=deg  TorqueActuationMode=NoTorque  MotionActuationMode=ComputedMotion  SensePosition=off  SenseVelocity=off  SenseAcceleration=off  SenseTorqueForce=off  SenseLowerLimitTorqueForce=off  SenseUpperLimitTorqueForce=off
  Actuator : Subsystem
  Base : Subsystem
  Inner Links : Subsystem
  "Inner Front Prismatic " : sm_lib/Joints/Prismatic Joint  JointMode=Normal  CompositeWrenchDir=FollowerOnBase  CompositeWrenchFrame=BaseFrame  SenseConstraintForce=off  SenseConstraintTorque=off  SenseTotalForce=off  SenseTotalTorque=off  PositionTargetSpecify=off  PositionTargetPriority=High  PositionTargetValue=0  PositionTargetValueUnits=m  VelocityTargetSpecify=off  VelocityTargetPriority=High  VelocityTargetValue=0  VelocityTargetValueUnits=m/s  EquilibriumPosition=0  EquilibriumPositionUnits=m  SpringStiffness=0  SpringStiffnessUnits=N/m  DampingCoefficient=0  DampingCoefficientUnits=N/(m/s)  LowerLimitSpecify=off  LowerLimitBound=-1  LowerLimitBoundUnits=m  LowerLimitStiffness=1e6  LowerLimitStiffnessUnits=N/m  LowerLimitDamping=1e3  LowerLimitDampingUnits=N/(m/s)  LowerLimitTransitionRegionWidth=1e-4  LowerLimitTransitionRegionWidthUnits=m  UpperLimitSpecify=off  UpperLimitBound=1  UpperLimitBoundUnits=m  UpperLimitStiffness=1e6  UpperLimitStiffnessUnits=N/m  UpperLimitDamping=1e3  UpperLimitDampingUnits=N/(m/s)  UpperLimitTransitionRegionWidth=1e-4  UpperLimitTransitionRegionWidthUnits=m  TorqueActuationMode=NoTorque  MotionActuationMode=ComputedMotion  SensePosition=off  SenseVelocity=off  SenseAcceleration=off  SenseTorqueForce=off  SenseLowerLimitTorqueForce=off  SenseUpperLimitTorqueForce=off
  Inner Rear Revolute : sm_lib/Joints/Revolute Joint  JointMode=Normal  CompositeWrenchDir=FollowerOnBase  CompositeWrenchFrame=BaseFrame  SenseConstraintForce=off  SenseConstraintTorque=off  SenseTotalForce=off  SenseTotalTorque=off  PositionTargetSpecify=off  PositionTargetPriority=Low  PositionTargetValue=15  PositionTargetValueUnits=deg  VelocityTargetSpecify=off  VelocityTargetPriority=High  VelocityTargetValue=0  VelocityTargetValueUnits=deg/s  EquilibriumPosition=0  EquilibriumPositionUnits=deg  SpringStiffness=0  SpringStiffnessUnits=N*m/deg  DampingCoefficient=0  DampingCoefficientUnits=N*m/(deg/s)  LowerLimitSpecify=off  LowerLimitBound=-90  LowerLimitBoundUnits=deg  LowerLimitStiffness=1e4  LowerLimitStiffnessUnits=N*m/deg  LowerLimitDamping=10  LowerLimitDampingUnits=N*m/(deg/s)  LowerLimitTransitionRegionWidth=0.1  LowerLimitTransitionRegionWidthUnits=deg  UpperLimitSpecify=off  UpperLimitBound=90  UpperLimitBoundUnits=deg  UpperLimitStiffness=1e4  UpperLimitStiffnessUnits=N*m/deg  UpperLimitDamping=10  UpperLimitDampingUnits=N*m/(deg/s)  UpperLimitTransitionRegionWidth=0.1  UpperLimitTransitionRegionWidthUnits=deg  TorqueActuationMode=NoTorque  MotionActuationMode=ComputedMotion  SensePosition=off  SenseVelocity=off  SenseAcceleration=off  SenseTorqueForce=off  SenseLowerLimitTorqueForce=off  SenseUpperLimitTorqueForce=off
  Outer Links : Subsystem
  "Outer Front Prismatic " : sm_lib/Joints/Prismatic Joint  JointMode=Normal  CompositeWrenchDir=FollowerOnBase  CompositeWrenchFrame=BaseFrame  SenseConstraintForce=off  SenseConstraintTorque=off  SenseTotalForce=off  SenseTotalTorque=off  PositionTargetSpecify=off  PositionTargetPriority=High  PositionTargetValue=0  PositionTargetValueUnits=m  VelocityTargetSpecify=off  VelocityTargetPriority=High  VelocityTargetValue=0  VelocityTargetValueUnits=m/s  EquilibriumPosition=0  EquilibriumPositionUnits=m  SpringStiffness=0  SpringStiffnessUnits=N/m  DampingCoefficient=0  DampingCoefficientUnits=N/(m/s)  LowerLimitSpecify=off  LowerLimitBound=-1  LowerLimitBoundUnits=m  LowerLimitStiffness=1e6  LowerLimitStiffnessUnits=N/m  LowerLimitDamping=1e3  LowerLimitDampingUnits=N/(m/s)  LowerLimitTransitionRegionWidth=1e-4  LowerLimitTransitionRegionWidthUnits=m  UpperLimitSpecify=off  UpperLimitBound=1  UpperLimitBoundUnits=m  UpperLimitStiffness=1e6  UpperLimitStiffnessUnits=N/m  UpperLimitDamping=1e3  UpperLimitDampingUnits=N/(m/s)  UpperLimitTransitionRegionWidth=1e-4  UpperLimitTransitionRegionWidthUnits=m  TorqueActuationMode=NoTorque  MotionActuationMode=ComputedMotion  SensePosition=off  SenseVelocity=off  SenseAcceleration=off  SenseTorqueForce=off  SenseLowerLimitTorqueForce=off  SenseUpperLimitTorqueForce=off
  Outer Rear Revolute : sm_lib/Joints/Revolute Joint  JointMode=Normal  CompositeWrenchDir=FollowerOnBase  CompositeWrenchFrame=BaseFrame  SenseConstraintForce=off  SenseConstraintTorque=off  SenseTotalForce=off  SenseTotalTorque=off  PositionTargetSpecify=off  PositionTargetPriority=Low  PositionTargetValue=-15  PositionTargetValueUnits=deg  VelocityTargetSpecify=off  VelocityTargetPriority=High  VelocityTargetValue=0  VelocityTargetValueUnits=deg/s  EquilibriumPosition=0  EquilibriumPositionUnits=deg  SpringStiffness=0  SpringStiffnessUnits=N*m/deg  DampingCoefficient=0  DampingCoefficientUnits=N*m/(deg/s)  LowerLimitSpecify=off  LowerLimitBound=-90  LowerLimitBoundUnits=deg  LowerLimitStiffness=1e4  LowerLimitStiffnessUnits=N*m/deg  LowerLimitDamping=10  LowerLimitDampingUnits=N*m/(deg/s)  LowerLimitTransitionRegionWidth=0.1  LowerLimitTransitionRegionWidthUnits=deg  UpperLimitSpecify=off  UpperLimitBound=90  UpperLimitBoundUnits=deg  UpperLimitStiffness=1e4  UpperLimitStiffnessUnits=N*m/deg  UpperLimitDamping=10  UpperLimitDampingUnits=N*m/(deg/s)  UpperLimitTransitionRegionWidth=0.1  UpperLimitTransitionRegionWidthUnits=deg  TorqueActuationMode=NoTorque  MotionActuationMode=ComputedMotion  SensePosition=off  SenseVelocity=off  SenseAcceleration=off  SenseTorqueForce=off  SenseLowerLimitTorqueForce=off  SenseUpperLimitTorqueForce=off
  Revolute Links Ctr : sm_lib/Joints/Revolute Joint  JointMode=Normal  CompositeWrenchDir=FollowerOnBase  CompositeWrenchFrame=BaseFrame  SenseConstraintForce=off  SenseConstraintTorque=off  SenseTotalForce=off  SenseTotalTorque=off  PositionTargetSpecify=on  PositionTargetPriority=Low  PositionTargetValue=-2*Scissor_Lift_Param.Initial_Angle  PositionTargetValueUnits=deg  VelocityTargetSpecify=off  VelocityTargetPriority=High  VelocityTargetValue=0  VelocityTargetValueUnits=deg/s  EquilibriumPosition=0  EquilibriumPositionUnits=deg  SpringStiffness=0  SpringStiffnessUnits=N*m/deg  DampingCoefficient=0  DampingCoefficientUnits=N*m/(deg/s)  LowerLimitSpecify=off  LowerLimitBound=-90  LowerLimitBoundUnits=deg  LowerLimitStiffness=1e4  LowerLimitStiffnessUnits=N*m/deg  LowerLimitDamping=10  LowerLimitDampingUnits=N*m/(deg/s)  LowerLimitTransitionRegionWidth=0.1  LowerLimitTransitionRegionWidthUnits=deg  UpperLimitSpecify=off  UpperLimitBound=90  UpperLimitBoundUnits=deg  UpperLimitStiffness=1e4  UpperLimitStiffnessUnits=N*m/deg  UpperLimitDamping=10  UpperLimitDampingUnits=N*m/(deg/s)  UpperLimitTransitionRegionWidth=0.1  UpperLimitTransitionRegionWidthUnits=deg  TorqueActuationMode=NoTorque  MotionActuationMode=ComputedMotion  SensePosition=off  SenseVelocity=off  SenseAcceleration=off  SenseTorqueForce=off  SenseLowerLimitTorqueForce=off  SenseUpperLimitTorqueForce=off
  Upper Platform : Subsystem
  R : PMIOPort  Side=Left
  C : PMIOPort  Port=2  Side=Left
  connections:
  Act Base Revolute/LConn1 -- Base/RConn2 -- Outer Rear Revolute/LConn1
  Inner Links/RConn1 -- "Inner Front Prismatic "/LConn1
  Base/RConn1 -- "Inner Front Prismatic "/RConn1
  Upper Platform/LConn2 -- "Outer Front Prismatic "/RConn1
  "Outer Front Prismatic "/LConn1 -- Outer Links/RConn2
  Inner Rear Revolute/LConn1 -- Upper Platform/LConn1
  Inner Links/LConn1 -- Inner Rear Revolute/RConn1
  Outer Rear Revolute/RConn1 -- Outer Links/LConn1
  Revolute Links Ctr/RConn1 -- Outer Links/RConn1
  Revolute Links Ctr/LConn1 -- Inner Links/LConn2
  Actuator/RConn1 -- Act Link Revolute/RConn1
  Act Link Revolute/LConn1 -- Inner Links/RConn2
  Actuator/LConn1 -- Act Base Revolute/RConn1
  C/RConn1 -- Actuator/LConn2
  R/RConn1 -- Actuator/RConn2

== system XFLUID04_reference/Load/Simple ==
  Gravity : fl_lib/Physical Signals/Sources/PS Constant  constant=9.81*Scissor_Lift_Param.Load.Mass
  Ideal Force Source : fl_lib/Mechanical/Mechanical Sources/Ideal Force Source
  Mass : fl_lib/Mechanical/Translational Elements/Mass  mass=Scissor_Lift_Param.Load.Mass kg  num_ports=foundation.enum.numPorts2.one  v_specify=on  v_priority=High  v=0 m/s  v_nominal_specify=off  v_nominal_value=1  v_nominal_unit=m/s  f_specify=off  f_priority=High  f=0 N  f_nominal_specify=off  f_nominal_value=1  f_nominal_unit=N
  Translational Damper : fl_lib/Mechanical/Translational Elements/Translational Damper  D=Scissor_Lift_Param.Actuator.Damping N/(m/s)  v_specify=off  v_priority=High  v=0 m/s  v_nominal_specify=off  v_nominal_value=1  v_nominal_unit=m/s  f_specify=off  f_priority=High  f=0 N  f_nominal_specify=off  f_nominal_value=1  f_nominal_unit=N
  R : PMIOPort  Side=Left
  C : PMIOPort  Port=2  Side=Left
  connections:
  Gravity/RConn1 -- Ideal Force Source/RConn1
  Ideal Force Source/RConn2 -- C/RConn1 -- Translational Damper/RConn1
  Mass/LConn1 -- Ideal Force Source/LConn1 -- R/RConn1 -- Translational Damper/LConn1

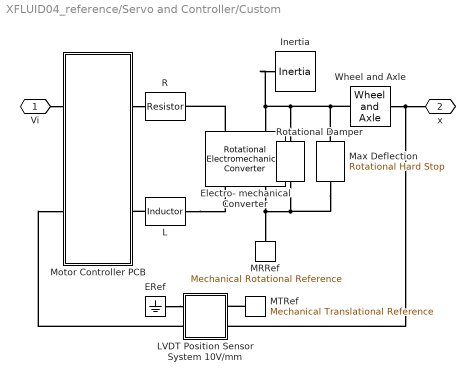
== system XFLUID04_reference/Servo and Controller/Custom ==
  ERef : fl_lib/Electrical/Electrical Elements/Electrical Reference
  Electro- mechanical Converter : fl_lib/Electrical/Electrical Elements/Rotational Electromechanical Converter  K=Kt V/(rad/s)  i_specify=off  i_priority=None  i=0 A  i_nominal_specify=off  i_nominal_value=1  i_nominal_unit=A  v_specify=off  v_priority=None  v=0 V  v_nominal_specify=off  v_nominal_value=1  v_nominal_unit=V  t_specify=off  t_priority=None  t=0 N*m  t_nominal_specify=off  t_nominal_value=1  t_nominal_unit=N*m  w_specify=off  w_priority=None  w=0 rad/s  w_nominal_specify=off  w_nominal_value=1  w_nominal_unit=rad/s
  Inertia : fl_lib/Mechanical/Rotational Elements/Inertia  inertia=J kg*m^2  num_ports=foundation.enum.numPorts2.one  w_specify=on  w_priority=High  w=0 rad/s  w_nominal_specify=off  w_nominal_value=1  w_nominal_unit=rad/s  t_specify=off  t_priority=None  t=0 N*m  t_nominal_specify=off  t_nominal_value=1  t_nominal_unit=N*m
  L : fl_lib/Electrical/Electrical Elements/Inductor  l=L H  r=0 Ohm  g=1e-09 1/Ohm  i_specify=off  i_priority=High  i=0 A  i_nominal_specify=off  i_nominal_value=1  i_nominal_unit=A  v_specify=off  v_priority=High  v=0 V  v_nominal_specify=off  v_nominal_value=1  v_nominal_unit=V  i_L_specify=on  i_L_priority=High  i_L=0 A  i_L_nominal_specify=off  i_L_nominal_value=1  i_L_nominal_unit=A
  LVDT Position Sensor System 10V/mm : Subsystem
  MRRef : fl_lib/Mechanical/Rotational Elements/Mechanical Rotational Reference
  MTRef : fl_lib/Mechanical/Translational Elements/Mechanical Translational Reference
  Max Deflection : fl_lib/Mechanical/Rotational Elements/Rotational Hard Stop  upper_bnd=x_max*1e-3/G rad  lower_bnd=-x_max*1e-3/G rad  model=3  stiff_up=1e+06 N*m/rad  stiff_low=1e+06 N*m/rad  D_up=0.05 N*m/(rad/s)  D_low=0.05 N*m/(rad/s)  transition=0.001 rad  coeff_rest=0.7  w_tol=0.1 rad/s  trq_tol=0.001 N*m  w_specify=off  w_priority=None  w=0 rad/s  w_nominal_specify=off  w_nominal_value=1  w_nominal_unit=rad/s  t_specify=off  t_priority=None  t=0 N*m  t_nominal_specify=off  t_nominal_value=1  t_nominal_unit=N*m  phi_specify=on  phi_priority=High  phi=0 rad  phi_nominal_specify=off  phi_nominal_value=1  phi_nominal_unit=rad  M_specify=off  M_priority=None  M=0
  Motor Controller PCB : Subsystem
  R : fl_lib/Electrical/Electrical Elements/Resistor  Tag=Factory Generic  R=R Ohm  i_specify=off  i_priority=High  i=0 A  i_nominal_specify=off  i_nominal_value=1  i_nominal_unit=A  v_specify=off  v_priority=High  v=0 V  v_nominal_specify=off  v_nominal_value=1  v_nominal_unit=V
  Rotational Damper : fl_lib/Mechanical/Rotational Elements/Rotational Damper  D=lambda N*m/(rad/s)  w_specify=off  w_priority=None  w=0 rad/s  w_nominal_specify=off  w_nominal_value=1  w_nominal_unit=rad/s  t_specify=off  t_priority=None  t=0 N*m  t_nominal_specify=off  t_nominal_value=1  t_nominal_unit=N*m
  Wheel and Axle : fl_lib/Mechanical/Mechanisms/Wheel and Axle  R=G m  or=1  t_specify=off  t_priority=High  t=0 N*m  t_nominal_specify=off  t_nominal_value=1  t_nominal_unit=N*m  f_specify=off  f_priority=High  f=0 N  f_nominal_specify=off  f_nominal_value=1  f_nominal_unit=N
  Vi : PMIOPort  Side=Left
  x : PMIOPort  Port=2  Side=Right
  connections:
  LVDT Position Sensor System 10V/mm/RConn2 -- Motor Controller PCB/LConn2
  ERef/LConn1 -- LVDT Position Sensor System 10V/mm/RConn1
  Vi/RConn1 -- Motor Controller PCB/LConn1
  Motor Controller PCB/RConn1 -- R/LConn1
  Electro- mechanical Converter/LConn1 -- R/RConn1
  Max Deflection/RConn1 -- Electro- mechanical Converter/RConn2 -- MRRef/LConn1 -- Rotational Damper/RConn1
  Inertia/LConn1 -- Max Deflection/LConn1 -- Wheel and Axle/LConn1 -- Rotational Damper/LConn1 -- Electro- mechanical Converter/LConn2
  L/LConn1 -- Motor Controller PCB/RConn2
  L/RConn1 -- Electro- mechanical Converter/RConn1
  LVDT Position Sensor System 10V/mm/LConn2 -- Wheel and Axle/RConn1 -- x/RConn1
  MTRef/LConn1 -- LVDT Position Sensor System 10V/mm/LConn1
